simulink model "afe_dqctrl_inv_psm"  (R2026a)
settings: Solver=ode23t  StopTime=simlength  FixedStep=tc  MaxStep=glb_time.tc  RelTol=1e-4
values from neighbouring files (symbols this model uses):
  afe_ctrl = ctrl_afe_setup(glb_time.ts_afe, grid_emu.omega_grid_nom)    [init_model.m]
  afe_pwm_phase_shift_mod1 = 0    [init_model.m]
  CTRPIFF_CLIP_RELEASE = 0.001    [init_model.m]
  filters = setup_global_filters(glb_time.ts_afe, glb_time.ts_inv, glb_time.ts_dab, glb_time.tc)    [init_model.m]
  glb_time = timing_setup(fpwm_afe, trgo_afe, fpwm_inv, trgo_inv, fpwm_single_phase_inv, trgo_single_phase_inv, fpwm_dab, trgo_dab,      fpwm_psfbc, trgo_psfbc, fpwm_isop_rail, trgo_isop_rail, fpwm_cllc, trgo_cllc, t_measure, tc_factor, tc_decimation, delay_pwm, dead_time_afe,      dead_time_inv, dead_time_single_phase_inv, dead_time_dab, dead_time_psfbc, dead_time_isop_rail, dead_time_cllc)    [init_model.m]
  grid_emu = grid_three_phase_emulator('Dyn11', delta_star, grid_nominal_power, application_voltage, us1, us2, fgrid,                  eq_grid_inductance, eq_grid_resistance, eta, ucc, i1m, p_iron, n1, n2, core_area, core_length, mur,                  up_xi_pu_ref, up_eta_pu_ref, un_xi_pu_ref, un_eta_pu_ref)    [init_model.m]
  heatsink = liquid_cooled_plate_2kw_setup(weight, no_weight, cp_al, heat_capacity_hs, thermal_conductivity_al,      Rth_switch_HA, Rth_mosfet_HA, Rth_diode_HA, Tambient, DThs_init)    [init_model.m]
  inv_pwm_phase_shift_mod1 = 0    [init_model.m]
  ki_align = 18    [init_model.m]
  kp_align = 0.25    [init_model.m]
  lim_down_align = -0.05    [init_model.m]
  lim_up_align = 0.05    [init_model.m]
  omega_m_sim = psm.omega_m_bez    [init_model.m]
  psm = psm_calculus()    [init_model.m]
  psm_ctrl = ctrl_pmsm_setup(glb_time.ts_inv, psm.omega_bez, u_psm_scale, psm.Jm_norm)    [init_model.m]
  simlength = 1.75    [init_model.m]
  Tambient = 40    [init_model.m]
  time_gain_afe_module_1 = 1.0002    [init_model.m]
  time_gain_inv_module_2 = 1.001    [init_model.m]
  time_start_motor_control = 0.25    [init_model.m]
  torque_overload_factor = 1.15    [init_model.m]
  u_cm_comp_mod1 = 0    [init_model.m]
  u_psm_scale_ekf = sqrt(3)/2 * 2/3 * hwdata.inv.udc_nom/psm.ubez    [init_model.m]
undefined symbols (not defined in the file or in its folder): hwdata, igbt, magnitude, omega_m_bez, rpm_base, torque_base
libraries: fl_lib x99, nesl_utility x96, igbt_simple_lib x12, single_phase_transformer_lib x3, threephase_inductor_lib x2, dclink_for_two_levels x2, three_phase_pwm_modulator x2, cstblocks_lti x2, discrete_time_low_pass_filter x1, lithium_ion_battery x1, three_phase_voltage_with_frt_emulator x1, simple_flexible_shaft x1
(part 7 of 9)

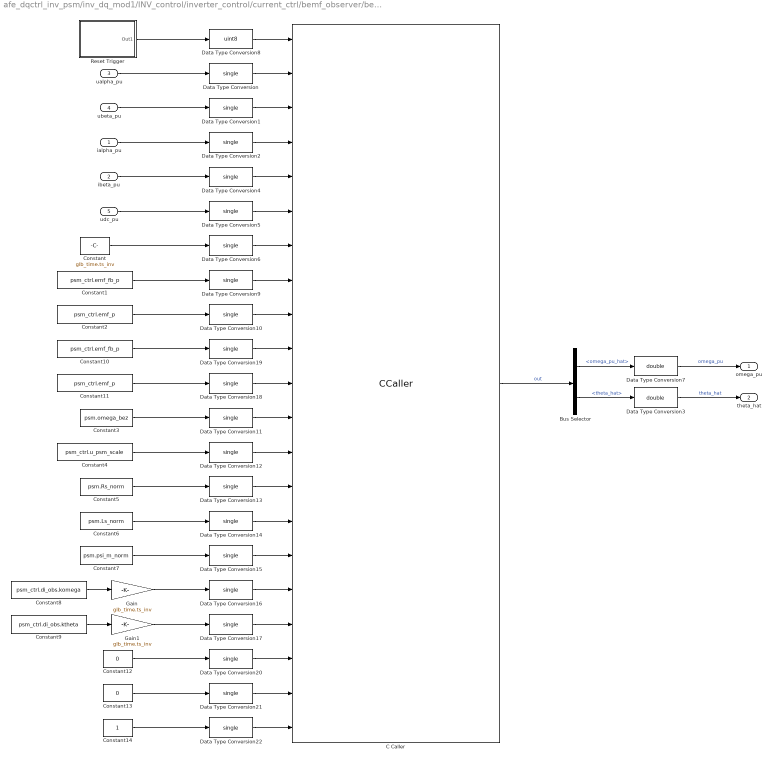
== system afe_dqctrl_inv_psm/inv_dq_mod1/INV_control/inverter_control/current_ctrl/bemf_observer/bemf_observer_ccaller ==
  ialpha_pu : Inport
  ibeta_pu : Inport  Port=2
  ualpha_pu : Inport  Port=3
  ubeta_pu : Inport  Port=4
  udc_pu : Inport  Port=5
  Bus Selector : BusSelector  OutputSignals=omega_pu_hat,theta_hat
  C Caller : CCaller  FunctionName=bemf_obsv_process_simulink  PortSpecificationStruct="%)30     .    N\"8   8    (     @         %    \"    !8    !     0         %  0 \"0    $    _    07)G3F%M90  4&]R=$YA;64 4V-O<&4     26YD97@     5'EP90      4VEZ90      27-';&]B86P   X    P    !@    @    $          4    (     0    ,    !         !   P!O=70 #@   #     &    \"     0         !0    @    !     P    $         $  # &]U=  .    .     8    (    !          %    \"     $    &     0         0  ...(+12985 chars)"
  Constant : Constant  Value=glb_time.ts_inv
  Constant1 : Constant  Value=psm_ctrl.emf_fb_p
  Constant10 : Constant  Value=psm_ctrl.emf_fb_p
  Constant11 : Constant  Value=psm_ctrl.emf_p
  Constant12 : Constant  Value=0
  Constant13 : Constant  Value=0
  Constant14 : Constant
  Constant2 : Constant  Value=psm_ctrl.emf_p
  Constant3 : Constant  Value=psm.omega_bez
  Constant4 : Constant  Value=psm_ctrl.u_psm_scale
  Constant5 : Constant  Value=psm.Rs_norm
  Constant6 : Constant  Value=psm.Ls_norm
  Constant7 : Constant  Value=psm.psi_m_norm
  Constant8 : Constant  Value=psm_ctrl.di_obs.komega
  Constant9 : Constant  Value=psm_ctrl.di_obs.ktheta
  Data Type Conversion{,1..2,4..6,9..22} (20 alike) : DataTypeConversion  OutDataTypeStr=single  SaturateOnIntegerOverflow=off  RndMeth=Floor
  Data Type Conversion3 : DataTypeConversion  OutDataTypeStr=double  SaturateOnIntegerOverflow=off  RndMeth=Floor
  Data Type Conversion7 : DataTypeConversion  OutDataTypeStr=double  SaturateOnIntegerOverflow=off  RndMeth=Floor
  Data Type Conversion8 : DataTypeConversion  OutDataTypeStr=uint8  SaturateOnIntegerOverflow=off  RndMeth=Floor
  Gain : Gain  Gain=glb_time.ts_inv
  Gain1 : Gain  Gain=glb_time.ts_inv
  Reset Trigger : Subsystem
  omega_pu : Outport
  theta_hat : Outport  Port=2
  wires:
  Data Type Conversion5/1 -> C Caller/6
  Data Type Conversion/1 -> C Caller/2
  C Caller/1 -> Bus Selector/1  "out"
  Data Type Conversion1/1 -> C Caller/3
  Data Type Conversion4/1 -> C Caller/5
  Data Type Conversion2/1 -> C Caller/4
  Data Type Conversion6/1 -> C Caller/7
  Bus Selector/2 -> Data Type Conversion3/1  "<theta_hat>"
  Bus Selector/1 -> Data Type Conversion7/1  "<omega_pu_hat>"
  Data Type Conversion7/1 -> omega_pu/1  "omega_pu"
  Data Type Conversion3/1 -> theta_hat/1  "theta_hat"
  Data Type Conversion8/1 -> C Caller/1
  Data Type Conversion9/1 -> C Caller/8
  Data Type Conversion10/1 -> C Caller/9
  Data Type Conversion19/1 -> C Caller/10
  Data Type Conversion18/1 -> C Caller/11
  Data Type Conversion11/1 -> C Caller/12
  Data Type Conversion12/1 -> C Caller/13
  Data Type Conversion13/1 -> C Caller/14
  Data Type Conversion14/1 -> C Caller/15
  Data Type Conversion15/1 -> C Caller/16
  Data Type Conversion16/1 -> C Caller/17
  Data Type Conversion17/1 -> C Caller/18
  Data Type Conversion20/1 -> C Caller/19
  Data Type Conversion21/1 -> C Caller/20
  Data Type Conversion22/1 -> C Caller/21
  Constant14/1 -> Data Type Conversion22/1
  Constant13/1 -> Data Type Conversion21/1
  Constant12/1 -> Data Type Conversion20/1
  Constant9/1 -> Gain1/1
  Constant8/1 -> Gain/1
  Constant7/1 -> Data Type Conversion15/1
  Constant6/1 -> Data Type Conversion14/1
  Constant5/1 -> Data Type Conversion13/1
  Constant4/1 -> Data Type Conversion12/1
  Constant3/1 -> Data Type Conversion11/1
  Constant11/1 -> Data Type Conversion18/1
  Constant10/1 -> Data Type Conversion19/1
  Constant2/1 -> Data Type Conversion10/1
  Constant1/1 -> Data Type Conversion9/1
  Constant/1 -> Data Type Conversion6/1
  ibeta_pu/1 -> Data Type Conversion4/1
  ialpha_pu/1 -> Data Type Conversion2/1
  ubeta_pu/1 -> Data Type Conversion1/1
  ualpha_pu/1 -> Data Type Conversion/1
  Reset Trigger/1(Out1) -> Data Type Conversion8/1
  udc_pu/1 -> Data Type Conversion5/1
  Gain/1 -> Data Type Conversion16/1
  Gain1/1 -> Data Type Conversion17/1

== system afe_dqctrl_inv_psm/inv_dq_mod1/INV_control/inverter_control/current_ctrl/current_ctrl/MTPA _mod1 ==
  iq_ref : Inport
  Gain1 : Gain  Gain=1/(psm.Ld_norm - psm.Lq_norm)/2
  Gain2 : Gain  Gain=1/(psm.Ld_norm - psm.Lq_norm)/2
  Gain3 : Gain  Gain=-1
  Math Function1 : Math  Operator=magnitude^2  SignedPower=on
  Math Function4 : Math  Operator=magnitude^2  SignedPower=on
  Sqrt : Sqrt
  Sum : Sum  Inputs=|++
  Sum1 : Sum  Inputs=|-+
  id_ref_pu < x < 0 : Saturate  UpperLimit=0  LowerLimit=-psm_ctrl.id_lim
  Id_ref_mtpa : Outport  VectorParamsAs1DForOutWhenUnconnected=off
  wires:
  Sum1/1 -> Gain3/1
  id_ref_pu < x < 0/1 -> Id_ref_mtpa/1
  Math Function4/1 -> Sum/1
  Math Function1/1 -> Sum/2
  Gain1/1 -> Math Function4/1
  Sum/1 -> Sqrt/1
  Sqrt/1 -> Sum1/2
  iq_ref/1 -> Math Function1/1
  Gain2/1 -> Sum1/1
  [motor_speed_pu_ctrl_mod1] -> Gain1/1, Gain2/1
  Gain3/1 -> id_ref_pu < x < 0/1

== system afe_dqctrl_inv_psm/inv_dq_mod1/INV_control/inverter_control/current_ctrl/current_ctrl/dq_pi_with_vector_antiwindup mod1 ==
  id_ref : Inport
  id : Inport  Port=2
  iq_ref : Inport  Port=3
  iq : Inport  Port=4
  udc_pu : Inport  Port=5
  Variant Source : VariantSource  VariantControls={use_current_controller_from_simulink_module_1 == 1, use_current_controller_from_ccaller_module_1 == 1}
  Variant Source1 : VariantSource  VariantControls={use_current_controller_from_simulink_module_1 == 1, use_current_controller_from_ccaller_module_1 == 1}
  dq_vector_pi : Subsystem
  dq_vector_pi_ccaller : Subsystem
  simulink/Ccaller VectorPI : Scope  NumInputPorts=2
      settings: ActiveDisplayYMinimum=-0.12579688616096973  ActiveDisplayYMaximum=0.43534495122730732
  ctrl_d_u : Outport
  ctrl_q_u : Outport  Port=2
  wires:
  id/1 -> dq_vector_pi_ccaller/1(id), dq_vector_pi/1(id)  "id"
  id_ref/1 -> dq_vector_pi_ccaller/2(id_ref), dq_vector_pi/2(id_ref)  "id_ref"
  iq/1 -> dq_vector_pi_ccaller/3(iq), dq_vector_pi/3(iq)  "iq"
  iq_ref/1 -> dq_vector_pi_ccaller/4(iq_ref), dq_vector_pi/4(iq_ref)  "iq_ref"
  dq_vector_pi/1(md_sat) -> Variant Source/1
  dq_vector_pi_ccaller/2(uq_ctrl_out) -> Variant Source1/2
  dq_vector_pi/2(mq_sat) -> Variant Source1/1
  dq_vector_pi_ccaller/1(ud_ctrl_out) -> Variant Source/2
  Variant Source/1 -> ctrl_d_u/1, simulink/Ccaller VectorPI/1  "ctrl_d_u"
  Variant Source1/1 -> simulink/Ccaller VectorPI/2, ctrl_q_u/1  "ctrl_q_u"
  udc_pu/1 -> dq_vector_pi_ccaller/5(udc_pu)

== system afe_dqctrl_inv_psm/inv_dq_mod1/INV_control/inverter_control/current_ctrl/current_ctrl/id_ref _mod1 ==
  id_mtpa : Inport
  Constant : Constant  Value=0
  Variant Source : VariantSource  VariantControls={use_mtpa == 1, use_mtpa == 0}
  id_ref : Outport
  wires:
  Variant Source/1 -> id_ref/1
  id_mtpa/1 -> Variant Source/1
  Constant/1 -> Variant Source/2

== system afe_dqctrl_inv_psm/inv_dq_mod1/INV_control/inverter_control/current_ctrl/current_ctrl/output voltage transformation ==
  Unit Delay2 : UnitDelay  SampleTime=-1
  Unit Delay3 : UnitDelay  SampleTime=-1
  dq2alphabeta : MATLAB Function  TreatAsAtomicUnit=on
  tag scope: ualpha_pu_mod1=scoped, ubeta_pu_mod1=scoped
  wires:
  [ud_pu_mod1] -> dq2alphabeta/1(d)
  [uq_pu_mod1] -> dq2alphabeta/2(q)
  Unit Delay2/1 -> [ualpha_pu_mod1]
  dq2alphabeta/2(beta) -> Unit Delay3/1
  Unit Delay3/1 -> [ubeta_pu_mod1]
  dq2alphabeta/1(alpha) -> Unit Delay2/1
  [motor_phase_ctrl_mod1] -> dq2alphabeta/3(gamma)

== system afe_dqctrl_inv_psm/inv_dq_mod1/INV_control/inverter_control/phase_compensation_1/alignment_ctrl/pi ==
  u_ref : Inport
  u : Inport  Port=2
  1/Ti : Gain  Gain=kp  SaturateOnIntegerOverflow=on  OutDataTypeStr=Inherit: Same as input  ParamDataTypeStr=Inherit: Same as input
  Saturation : Saturate  UpperLimit=lim_up  LowerLimit=lim_down
  Sum1 : Sum  Inputs=+++  SaturateOnIntegerOverflow=on
  Sum2 : Sum  Inputs=-+  SaturateOnIntegerOverflow=on
  Sum3 : Sum  Inputs=-+  SaturateOnIntegerOverflow=on
  Unit Delay4 : UnitDelay  SampleTime=-1
  kp : Gain  Gain=ki  SaturateOnIntegerOverflow=on  OutDataTypeStr=Inherit: Same as input  ParamDataTypeStr=Inherit: Same as input
  y : Outport
  wires:
  1/Ti/1 -> Sum1/1, Sum3/1
  kp/1 -> Sum1/2
  Sum3/1 -> Unit Delay4/1
  Unit Delay4/1 -> Sum1/3
  u_ref/1 -> Sum2/2
  u/1 -> Sum2/1
  Sum2/1 -> kp/1, 1/Ti/1
  Sum1/1 -> Saturation/1
  Saturation/1 -> Sum3/2, y/1

== system afe_dqctrl_inv_psm/inv_dq_mod1/inverter/inverter/three_phase_inverter_with_igbt_simple/three_phase_inverter_with_igbt_simple/igbt_simple_1 ==
  note: P_sw
  Capacitor : fl_lib/Electrical/Electrical Elements/Capacitor  c=Csnubber_m F  r=Rsnubber_m Ohm  g=0 1/Ohm  i_specify=off  i_priority=None  i=0 A  i_nominal_specify=off  i_nominal_value=1  i_nominal_unit=A  v_specify=off  v_priority=None  v=0 V  v_nominal_specify=off  v_nominal_value=1  v_nominal_unit=V  vc_specify=off  vc_priority=High  vc=0 V  vc_nominal_specify=off  vc_nominal_value=1  vc_nominal_unit=V
  IGBT_simple : Subsystem
      settings: PortSchema="{\"entries\":[{\"content\":{\"sides\":[{\"content\":{\"connectorIds\":[\"LConn1\"]},\"type\":\"ConnectorPlacement.EquallySpacedRectSide\",\"uuid\":\"c3d88d60-081d-4221-ab18-079856838dba\"},{\"content\":{\"side\":\"RIGHT\"},\"type\":\"ConnectorPlacement.EquallySpacedRectSide\",\"uuid\":\"76e7d76c-8b60-4107-8aac-a7654bd886e1\"},{\"content\":{\"connectorIds\":[\"LConn2\"],\"side\":\"TOP\"},\"type\":\"ConnectorPlacement.EquallySpacedRectSide\",\"uuid\":\"fbef57e1-7143-4076-ada8-0654b1d9ee0b\"},{\"content\":{\"connectorIds\":[\"RConn1\"],\"side\":\"BOTTOM\"},\"type\":\"ConnectorPlacement.EquallySpacedRectSide\",\"uuid\":\"f2fea5db-9515-452a-a480-7d54bae36c49\"}]},\"type\":\"ConnectorPlacement.EquallySpacedConnector\",\"uuid\":\"cddff0b8-236e-4840-ad87-03abcdd65fe7\"}],\"packageUris\":[\"http://schema.mathworks.com/mf0/Connector/R2020b\"],\"version\":\"1.0\"}"
  Voltage Sensor : fl_lib/Electrical/Electrical Sensors/Voltage Sensor
  uph : nesl_utility/PS-Simulink Converter  PhysicalDomain=network_engine_domain  SubClassName=ps_output  LeftPortType=input  RightPortType=output  PseudoPeriodic=off  Frequencies=[]  VectorFormat=1-D array  Unit=V  AffineConversion=off
  G : PMIOPort  Side=Left
  C : PMIOPort  Port=2  Side=Left
  E : PMIOPort  Port=3  Side=Right
  tag scope: igbt_voltage_Q1=scoped
  wires:
  uph/1 -> [igbt_voltage_Q1]  "uph"
  connections:
  G/RConn1 -- IGBT_simple/LConn1
  Voltage Sensor/RConn1 -- uph/LConn1
  Capacitor/LConn1 -- Voltage Sensor/LConn1 -- C/RConn1 -- IGBT_simple/LConn2
  Capacitor/RConn1 -- Voltage Sensor/RConn2 -- E/RConn1 -- IGBT_simple/RConn1

== system afe_dqctrl_inv_psm/inv_dq_mod1/inverter/inverter/three_phase_inverter_with_igbt_simple/three_phase_inverter_with_igbt_simple/igbt_simple_2 ==
  Capacitor : fl_lib/Electrical/Electrical Elements/Capacitor  c=Csnubber_m F  r=Rsnubber_m Ohm  g=0 1/Ohm  i_specify=off  i_priority=None  i=0 A  i_nominal_specify=off  i_nominal_value=1  i_nominal_unit=A  v_specify=off  v_priority=None  v=0 V  v_nominal_specify=off  v_nominal_value=1  v_nominal_unit=V  vc_specify=off  vc_priority=High  vc=0 V  vc_nominal_specify=off  vc_nominal_value=1  vc_nominal_unit=V
  IGBT_simple : Subsystem
      settings: PortSchema="{\"entries\":[{\"content\":{\"sides\":[{\"content\":{\"connectorIds\":[\"LConn1\"]},\"type\":\"ConnectorPlacement.EquallySpacedRectSide\",\"uuid\":\"c3d88d60-081d-4221-ab18-079856838dba\"},{\"content\":{\"side\":\"RIGHT\"},\"type\":\"ConnectorPlacement.EquallySpacedRectSide\",\"uuid\":\"76e7d76c-8b60-4107-8aac-a7654bd886e1\"},{\"content\":{\"connectorIds\":[\"LConn2\"],\"side\":\"TOP\"},\"type\":\"ConnectorPlacement.EquallySpacedRectSide\",\"uuid\":\"fbef57e1-7143-4076-ada8-0654b1d9ee0b\"},{\"content\":{\"connectorIds\":[\"RConn1\"],\"side\":\"BOTTOM\"},\"type\":\"ConnectorPlacement.EquallySpacedRectSide\",\"uuid\":\"f2fea5db-9515-452a-a480-7d54bae36c49\"}]},\"type\":\"ConnectorPlacement.EquallySpacedConnector\",\"uuid\":\"cddff0b8-236e-4840-ad87-03abcdd65fe7\"}],\"packageUris\":[\"http://schema.mathworks.com/mf0/Connector/R2020b\"],\"version\":\"1.0\"}"
  Voltage Sensor : fl_lib/Electrical/Electrical Sensors/Voltage Sensor
  uph : nesl_utility/PS-Simulink Converter  PhysicalDomain=network_engine_domain  SubClassName=ps_output  LeftPortType=input  RightPortType=output  PseudoPeriodic=off  Frequencies=[]  VectorFormat=1-D array  Unit=V  AffineConversion=off
  G : PMIOPort  Side=Left
  C : PMIOPort  Port=2  Side=Left
  E : PMIOPort  Port=3  Side=Right
  tag scope: igbt_voltage_Q2=scoped
  wires:
  uph/1 -> [igbt_voltage_Q2]  "uph"
  connections:
  Capacitor/RConn1 -- Voltage Sensor/RConn2 -- E/RConn1 -- IGBT_simple/RConn1
  Capacitor/LConn1 -- Voltage Sensor/LConn1 -- C/RConn1 -- IGBT_simple/LConn2
  Voltage Sensor/RConn1 -- uph/LConn1
  IGBT_simple/LConn1 -- G/RConn1

== system afe_dqctrl_inv_psm/inv_dq_mod1/inverter/inverter/three_phase_inverter_with_igbt_simple/three_phase_inverter_with_igbt_simple/igbt_simple_3 ==
  Capacitor : fl_lib/Electrical/Electrical Elements/Capacitor  c=Csnubber_m F  r=Rsnubber_m Ohm  g=0 1/Ohm  i_specify=off  i_priority=None  i=0 A  i_nominal_specify=off  i_nominal_value=1  i_nominal_unit=A  v_specify=off  v_priority=None  v=0 V  v_nominal_specify=off  v_nominal_value=1  v_nominal_unit=V  vc_specify=off  vc_priority=High  vc=0 V  vc_nominal_specify=off  vc_nominal_value=1  vc_nominal_unit=V
  IGBT_simple : Subsystem
      settings: PortSchema="{\"entries\":[{\"content\":{\"sides\":[{\"content\":{\"connectorIds\":[\"LConn1\"]},\"type\":\"ConnectorPlacement.EquallySpacedRectSide\",\"uuid\":\"c3d88d60-081d-4221-ab18-079856838dba\"},{\"content\":{\"side\":\"RIGHT\"},\"type\":\"ConnectorPlacement.EquallySpacedRectSide\",\"uuid\":\"76e7d76c-8b60-4107-8aac-a7654bd886e1\"},{\"content\":{\"connectorIds\":[\"LConn2\"],\"side\":\"TOP\"},\"type\":\"ConnectorPlacement.EquallySpacedRectSide\",\"uuid\":\"fbef57e1-7143-4076-ada8-0654b1d9ee0b\"},{\"content\":{\"connectorIds\":[\"RConn1\"],\"side\":\"BOTTOM\"},\"type\":\"ConnectorPlacement.EquallySpacedRectSide\",\"uuid\":\"f2fea5db-9515-452a-a480-7d54bae36c49\"}]},\"type\":\"ConnectorPlacement.EquallySpacedConnector\",\"uuid\":\"cddff0b8-236e-4840-ad87-03abcdd65fe7\"}],\"packageUris\":[\"http://schema.mathworks.com/mf0/Connector/R2020b\"],\"version\":\"1.0\"}"
  Voltage Sensor : fl_lib/Electrical/Electrical Sensors/Voltage Sensor
  uph : nesl_utility/PS-Simulink Converter  PhysicalDomain=network_engine_domain  SubClassName=ps_output  LeftPortType=input  RightPortType=output  PseudoPeriodic=off  Frequencies=[]  VectorFormat=1-D array  Unit=V  AffineConversion=off
  G : PMIOPort  Side=Left
  C : PMIOPort  Port=2  Side=Left
  E : PMIOPort  Port=3  Side=Right
  tag scope: igbt_voltage_Q3=scoped
  wires:
  uph/1 -> [igbt_voltage_Q3]  "uph"
  connections:
  IGBT_simple/LConn1 -- G/RConn1
  Voltage Sensor/RConn1 -- uph/LConn1
  Voltage Sensor/LConn1 -- Capacitor/LConn1 -- C/RConn1 -- IGBT_simple/LConn2
  Voltage Sensor/RConn2 -- Capacitor/RConn1 -- E/RConn1 -- IGBT_simple/RConn1

== system afe_dqctrl_inv_psm/inv_dq_mod1/inverter/inverter/three_phase_inverter_with_igbt_simple/three_phase_inverter_with_igbt_simple/igbt_simple_4 ==
  Capacitor : fl_lib/Electrical/Electrical Elements/Capacitor  c=Csnubber_m F  r=Rsnubber_m Ohm  g=0 1/Ohm  i_specify=off  i_priority=None  i=0 A  i_nominal_specify=off  i_nominal_value=1  i_nominal_unit=A  v_specify=off  v_priority=None  v=0 V  v_nominal_specify=off  v_nominal_value=1  v_nominal_unit=V  vc_specify=off  vc_priority=High  vc=0 V  vc_nominal_specify=off  vc_nominal_value=1  vc_nominal_unit=V
  IGBT_simple : Subsystem
      settings: PortSchema="{\"entries\":[{\"content\":{\"sides\":[{\"content\":{\"connectorIds\":[\"LConn1\"]},\"type\":\"ConnectorPlacement.EquallySpacedRectSide\",\"uuid\":\"c3d88d60-081d-4221-ab18-079856838dba\"},{\"content\":{\"side\":\"RIGHT\"},\"type\":\"ConnectorPlacement.EquallySpacedRectSide\",\"uuid\":\"76e7d76c-8b60-4107-8aac-a7654bd886e1\"},{\"content\":{\"connectorIds\":[\"LConn2\"],\"side\":\"TOP\"},\"type\":\"ConnectorPlacement.EquallySpacedRectSide\",\"uuid\":\"fbef57e1-7143-4076-ada8-0654b1d9ee0b\"},{\"content\":{\"connectorIds\":[\"RConn1\"],\"side\":\"BOTTOM\"},\"type\":\"ConnectorPlacement.EquallySpacedRectSide\",\"uuid\":\"f2fea5db-9515-452a-a480-7d54bae36c49\"}]},\"type\":\"ConnectorPlacement.EquallySpacedConnector\",\"uuid\":\"cddff0b8-236e-4840-ad87-03abcdd65fe7\"}],\"packageUris\":[\"http://schema.mathworks.com/mf0/Connector/R2020b\"],\"version\":\"1.0\"}"
  Voltage Sensor : fl_lib/Electrical/Electrical Sensors/Voltage Sensor
  uph : nesl_utility/PS-Simulink Converter  PhysicalDomain=network_engine_domain  SubClassName=ps_output  LeftPortType=input  RightPortType=output  PseudoPeriodic=off  Frequencies=[]  VectorFormat=1-D array  Unit=V  AffineConversion=off
  G : PMIOPort  Side=Left
  C : PMIOPort  Port=2  Side=Left
  E : PMIOPort  Port=3  Side=Right
  tag scope: igbt_voltage_Q4=scoped
  wires:
  uph/1 -> [igbt_voltage_Q4]  "uph"
  connections:
  Capacitor/RConn1 -- Voltage Sensor/RConn2 -- E/RConn1 -- IGBT_simple/RConn1
  Capacitor/LConn1 -- Voltage Sensor/LConn1 -- C/RConn1 -- IGBT_simple/LConn2
  Voltage Sensor/RConn1 -- uph/LConn1
  IGBT_simple/LConn1 -- G/RConn1

== system afe_dqctrl_inv_psm/inv_dq_mod1/inverter/inverter/three_phase_inverter_with_igbt_simple/three_phase_inverter_with_igbt_simple/igbt_simple_5 ==
  Capacitor : fl_lib/Electrical/Electrical Elements/Capacitor  c=Csnubber_m F  r=Rsnubber_m Ohm  g=0 1/Ohm  i_specify=off  i_priority=None  i=0 A  i_nominal_specify=off  i_nominal_value=1  i_nominal_unit=A  v_specify=off  v_priority=None  v=0 V  v_nominal_specify=off  v_nominal_value=1  v_nominal_unit=V  vc_specify=off  vc_priority=High  vc=0 V  vc_nominal_specify=off  vc_nominal_value=1  vc_nominal_unit=V
  IGBT_simple : Subsystem
      settings: PortSchema="{\"entries\":[{\"content\":{\"sides\":[{\"content\":{\"connectorIds\":[\"LConn1\"]},\"type\":\"ConnectorPlacement.EquallySpacedRectSide\",\"uuid\":\"c3d88d60-081d-4221-ab18-079856838dba\"},{\"content\":{\"side\":\"RIGHT\"},\"type\":\"ConnectorPlacement.EquallySpacedRectSide\",\"uuid\":\"76e7d76c-8b60-4107-8aac-a7654bd886e1\"},{\"content\":{\"connectorIds\":[\"LConn2\"],\"side\":\"TOP\"},\"type\":\"ConnectorPlacement.EquallySpacedRectSide\",\"uuid\":\"fbef57e1-7143-4076-ada8-0654b1d9ee0b\"},{\"content\":{\"connectorIds\":[\"RConn1\"],\"side\":\"BOTTOM\"},\"type\":\"ConnectorPlacement.EquallySpacedRectSide\",\"uuid\":\"f2fea5db-9515-452a-a480-7d54bae36c49\"}]},\"type\":\"ConnectorPlacement.EquallySpacedConnector\",\"uuid\":\"cddff0b8-236e-4840-ad87-03abcdd65fe7\"}],\"packageUris\":[\"http://schema.mathworks.com/mf0/Connector/R2020b\"],\"version\":\"1.0\"}"
  Voltage Sensor : fl_lib/Electrical/Electrical Sensors/Voltage Sensor
  uph : nesl_utility/PS-Simulink Converter  PhysicalDomain=network_engine_domain  SubClassName=ps_output  LeftPortType=input  RightPortType=output  PseudoPeriodic=off  Frequencies=[]  VectorFormat=1-D array  Unit=V  AffineConversion=off
  G : PMIOPort  Side=Left
  C : PMIOPort  Port=2  Side=Left
  E : PMIOPort  Port=3  Side=Right
  tag scope: igbt_voltage_Q5=scoped
  wires:
  uph/1 -> [igbt_voltage_Q5]  "uph"
  connections:
  IGBT_simple/LConn1 -- G/RConn1
  Voltage Sensor/RConn1 -- uph/LConn1
  Voltage Sensor/LConn1 -- Capacitor/LConn1 -- C/RConn1 -- IGBT_simple/LConn2
  Voltage Sensor/RConn2 -- Capacitor/RConn1 -- E/RConn1 -- IGBT_simple/RConn1

== system afe_dqctrl_inv_psm/inv_dq_mod1/inverter/inverter/three_phase_inverter_with_igbt_simple/three_phase_inverter_with_igbt_simple/igbt_simple_6 ==
  Capacitor : fl_lib/Electrical/Electrical Elements/Capacitor  c=Csnubber_m F  r=Rsnubber_m Ohm  g=0 1/Ohm  i_specify=off  i_priority=None  i=0 A  i_nominal_specify=off  i_nominal_value=1  i_nominal_unit=A  v_specify=off  v_priority=None  v=0 V  v_nominal_specify=off  v_nominal_value=1  v_nominal_unit=V  vc_specify=off  vc_priority=High  vc=0 V  vc_nominal_specify=off  vc_nominal_value=1  vc_nominal_unit=V
  IGBT_simple : Subsystem
      settings: PortSchema="{\"entries\":[{\"content\":{\"sides\":[{\"content\":{\"connectorIds\":[\"LConn1\"]},\"type\":\"ConnectorPlacement.EquallySpacedRectSide\",\"uuid\":\"c3d88d60-081d-4221-ab18-079856838dba\"},{\"content\":{\"side\":\"RIGHT\"},\"type\":\"ConnectorPlacement.EquallySpacedRectSide\",\"uuid\":\"76e7d76c-8b60-4107-8aac-a7654bd886e1\"},{\"content\":{\"connectorIds\":[\"LConn2\"],\"side\":\"TOP\"},\"type\":\"ConnectorPlacement.EquallySpacedRectSide\",\"uuid\":\"fbef57e1-7143-4076-ada8-0654b1d9ee0b\"},{\"content\":{\"connectorIds\":[\"RConn1\"],\"side\":\"BOTTOM\"},\"type\":\"ConnectorPlacement.EquallySpacedRectSide\",\"uuid\":\"f2fea5db-9515-452a-a480-7d54bae36c49\"}]},\"type\":\"ConnectorPlacement.EquallySpacedConnector\",\"uuid\":\"cddff0b8-236e-4840-ad87-03abcdd65fe7\"}],\"packageUris\":[\"http://schema.mathworks.com/mf0/Connector/R2020b\"],\"version\":\"1.0\"}"
  Voltage Sensor : fl_lib/Electrical/Electrical Sensors/Voltage Sensor
  uph : nesl_utility/PS-Simulink Converter  PhysicalDomain=network_engine_domain  SubClassName=ps_output  LeftPortType=input  RightPortType=output  PseudoPeriodic=off  Frequencies=[]  VectorFormat=1-D array  Unit=V  AffineConversion=off
  G : PMIOPort  Side=Left
  C : PMIOPort  Port=2  Side=Left
  E : PMIOPort  Port=3  Side=Right
  tag scope: igbt_voltage_Q6=scoped
  wires:
  uph/1 -> [igbt_voltage_Q6]  "uph"
  connections:
  Capacitor/RConn1 -- Voltage Sensor/RConn2 -- E/RConn1 -- IGBT_simple/RConn1
  Capacitor/LConn1 -- Voltage Sensor/LConn1 -- C/RConn1 -- IGBT_simple/LConn2
  Voltage Sensor/RConn1 -- uph/LConn1
  IGBT_simple/LConn1 -- G/RConn1

== system afe_dqctrl_inv_psm/inv_dq_mod1/inverter/inverter/three_phase_inverter_with_igbt_simple/three_phase_inverter_with_igbt_simple/module_1 ==
  Bus Creator : BusCreator  Inputs=18
  m : Outport
  wires:
  [diode_HA_temp_Q1] -> Bus Creator/8  "diode_HA_temp_Q1"
  [igbt_voltage_Q2] -> Bus Creator/10  "igbt_voltage_Q2"
  [igbt_voltage_Q1] -> Bus Creator/2  "igbt_voltage_Q1"
  [igbt_ploss_Q2] -> Bus Creator/9  "igbt_ploss_Q2"
  [igbt_current_Q2] -> Bus Creator/11  "igbt_current_Q2"
  [diode_ploss_Q1] -> Bus Creator/6  "diode_ploss_Q1"
  [diode_JH_temp_Q1] -> Bus Creator/7  "diode_JH_temp_Q1"
  [igbt_HA_temp_Q1] -> Bus Creator/5  "igbt_HA_temp_Q1"
  [igbt_ploss_Q1] -> Bus Creator/1  "igbt_ploss_Q1"
  [diode_JH_temp_Q2] -> Bus Creator/15  "diode_JH_temp_Q2"
  [diode_HA_temp_Q2] -> Bus Creator/16  "diode_HA_temp_Q2"
  [diode_ploss_Q2] -> Bus Creator/14  "diode_ploss_Q2"
  [igbt_HA_temp_Q2] -> Bus Creator/13  "igbt_HA_temp_Q2"
  [igbt_JH_temp_Q2] -> Bus Creator/12  "igbt_JH_temp_Q2"
  [igbt_JH_temp_Q1] -> Bus Creator/4  "igbt_JH_temp_Q1"
  [igbt_current_Q1] -> Bus Creator/3  "igbt_current_Q1"
  Bus Creator/1 -> m/1  "module_1"
  [diode_current_Q1] -> Bus Creator/17  "diode_current_Q1"
  [diode_current_Q2] -> Bus Creator/18  "diode_current_Q2"

== system afe_dqctrl_inv_psm/inv_dq_mod1/inverter/inverter/three_phase_inverter_with_igbt_simple/three_phase_inverter_with_igbt_simple/module_2 ==
  Bus Creator1 : BusCreator  Inputs=18
  m : Outport
  wires:
  [diode_HA_temp_Q4] -> Bus Creator1/16  "diode_HA_temp_Q4"
  [igbt_HA_temp_Q3] -> Bus Creator1/5  "igbt_HA_temp_Q3"
  [igbt_JH_temp_Q3] -> Bus Creator1/4  "igbt_JH_temp_Q3"
  [diode_ploss_Q3] -> Bus Creator1/6  "diode_ploss_Q3"
  [diode_JH_temp_Q4] -> Bus Creator1/15  "diode_JH_temp_Q4"
  [igbt_ploss_Q3] -> Bus Creator1/1  "igbt_ploss_Q3"
  [igbt_JH_temp_Q4] -> Bus Creator1/12  "igbt_JH_temp_Q4"
  [igbt_voltage_Q3] -> Bus Creator1/2  "igbt_voltage_Q3"
  [igbt_current_Q4] -> Bus Creator1/11  "igbt_current_Q4"
  [diode_HA_temp_Q3] -> Bus Creator1/8  "diode_HA_temp_Q3"
  [igbt_voltage_Q4] -> Bus Creator1/10  "igbt_voltage_Q4"
  [igbt_ploss_Q4] -> Bus Creator1/9  "igbt_ploss_Q4"
  [igbt_HA_temp_Q4] -> Bus Creator1/13  "igbt_HA_temp_Q4"
  [diode_JH_temp_Q3] -> Bus Creator1/7  "diode_JH_temp_Q3"
  [diode_ploss_Q4] -> Bus Creator1/14  "diode_ploss_Q4"
  [igbt_current_Q3] -> Bus Creator1/3  "igbt_current_Q3"
  Bus Creator1/1 -> m/1  "module_2"
  [diode_current_Q4] -> Bus Creator1/18  "diode_current_Q4"
  [diode_current_Q3] -> Bus Creator1/17  "diode_current_Q3"

== system afe_dqctrl_inv_psm/inv_dq_mod1/inverter/inverter/three_phase_inverter_with_igbt_simple/three_phase_inverter_with_igbt_simple/module_3 ==
  Bus Creator1 : BusCreator  Inputs=18
  m : Outport
  wires:
  [diode_ploss_Q6] -> Bus Creator1/14  "diode_ploss_Q6"
  [igbt_HA_temp_Q5] -> Bus Creator1/5  "igbt_HA_temp_Q5"
  [igbt_voltage_Q6] -> Bus Creator1/10  "igbt_voltage_Q6"
  [igbt_voltage_Q5] -> Bus Creator1/2  "igbt_voltage_Q5"
  [igbt_JH_temp_Q6] -> Bus Creator1/12  "igbt_JH_temp_Q6"
  [igbt_current_Q6] -> Bus Creator1/11  "igbt_current_Q6"
  [diode_JH_temp_Q6] -> Bus Creator1/15  "diode_JH_temp_Q6"
  [diode_HA_temp_Q5] -> Bus Creator1/8  "diode_HA_temp_Q5"
  [igbt_ploss_Q5] -> Bus Creator1/1  "igbt_ploss_Q5"
  [igbt_ploss_Q6] -> Bus Creator1/9  "igbt_ploss_Q6"
  [igbt_current_Q5] -> Bus Creator1/3  "igbt_current_Q5"
  [diode_JH_temp_Q5] -> Bus Creator1/7  "diode_JH_temp_Q5"
  [igbt_JH_temp_Q5] -> Bus Creator1/4  "igbt_JH_temp_Q5"
  [diode_HA_temp_Q6] -> Bus Creator1/16  "diode_HA_temp_Q6"
  [igbt_HA_temp_Q6] -> Bus Creator1/13  "igbt_HA_temp_Q6"
  [diode_ploss_Q5] -> Bus Creator1/6  "diode_ploss_Q5"
  Bus Creator1/1 -> m/1  "module_3"
  [diode_current_Q6] -> Bus Creator1/18  "diode_current_Q6"
  [diode_current_Q5] -> Bus Creator1/17  "diode_current_Q5"

== system afe_dqctrl_inv_psm/afe_dq_mod1/AFE_control/afe_control/acquisitions/phase_compensation_1/alignment_eval_afe1/pi ==
  u_ref : Inport
  u : Inport  Port=2
  1/Ti : Gain  Gain=kp  SaturateOnIntegerOverflow=on  OutDataTypeStr=Inherit: Same as input  ParamDataTypeStr=Inherit: Same as input
  Saturation : Saturate  UpperLimit=lim_up  LowerLimit=lim_down
  Sum1 : Sum  Inputs=+++  SaturateOnIntegerOverflow=on
  Sum2 : Sum  Inputs=-+  SaturateOnIntegerOverflow=on
  Sum3 : Sum  Inputs=-+  SaturateOnIntegerOverflow=on
  Unit Delay4 : UnitDelay  SampleTime=-1
  kp : Gain  Gain=ki  SaturateOnIntegerOverflow=on  OutDataTypeStr=Inherit: Same as input  ParamDataTypeStr=Inherit: Same as input
  y : Outport
  wires:
  1/Ti/1 -> Sum1/1, Sum3/1
  kp/1 -> Sum1/2
  Sum3/1 -> Unit Delay4/1
  Unit Delay4/1 -> Sum1/3
  u_ref/1 -> Sum2/2
  u/1 -> Sum2/1
  Sum2/1 -> kp/1, 1/Ti/1
  Sum1/1 -> Saturation/1
  Saturation/1 -> Sum3/2, y/1

== system afe_dqctrl_inv_psm/afe_dq_mod1/AFE_control/afe_control/grid_voltage_phase_lock_loops/FHT-PLL/pll_stageA/filter_and_transformation ==
  ug_a : Inport
  ug_b : Inport  Port=2
  ug_c : Inport  Port=3
  Bus Creator : BusCreator  Inputs=2
  Bus Creator1 : BusCreator  Inputs=3
  Bus Creator2 : BusCreator  Inputs=2
  Bus Creator3 : BusCreator  Inputs=3
  Bus Creator4 : BusCreator  Inputs=3
  FHTalpha : Subsystem
  FHTbeta : Subsystem
  FHTdqPLL : Scope  NumInputPorts=2
      settings: ActiveDisplayYMinimum=-1.5258214459194912  ActiveDisplayYMaximum=1.5258228058860459  DataLoggingVariableName=ScopeData12
  Gain : Gain  Gain=-1/2
  Gain1 : Gain  Gain=-1/2
  Sum : Sum  Inputs=|++
  Sum1 : Sum  Inputs=-+|
  To Workspace1 : ToWorkspace  VariableName=ugd_alpha_sim  SampleTime=-1
      settings: MaxDataPoints=glb_time.Ns_afe
  To Workspace2 : ToWorkspace  VariableName=ugd_beta_sim  SampleTime=-1
      settings: MaxDataPoints=glb_time.Ns_afe
  To Workspace3 : ToWorkspace  VariableName=u_fht_alpha_sim  SampleTime=-1
      settings: MaxDataPoints=glb_time.Ns_afe
  To Workspace4 : ToWorkspace  VariableName=v_fht_alpha_sim  SampleTime=-1
      settings: MaxDataPoints=glb_time.Ns_afe
  To Workspace5 : ToWorkspace  VariableName=u_fhtsr_alpha_sim  SampleTime=-1
      settings: MaxDataPoints=glb_time.Ns_afe
  To Workspace6 : ToWorkspace  VariableName=u_fhtsr_beta_sim  SampleTime=-1
      settings: MaxDataPoints=glb_time.Ns_afe
  To Workspace7 : ToWorkspace  VariableName=u_fht_beta_sim  SampleTime=-1
      settings: MaxDataPoints=glb_time.Ns_afe
  To Workspace8 : ToWorkspace  VariableName=v_fht_beta_sim  SampleTime=-1
      settings: MaxDataPoints=glb_time.Ns_afe
  To Workspace9 : ToWorkspace  VariableName=ugd_abc_grid_sim  SampleTime=-1
      settings: MaxDataPoints=glb_time.Ns_afe
  abc2alphabeta : MATLAB Function  TreatAsAtomicUnit=on
  grid_voltages : Scope  NumInputPorts=3
      settings: ActiveDisplayYMinimum=-1.3618303835391998  ActiveDisplayYMaximum=1.3331545889377594  DataLoggingVariableName=ScopeData13
  ug_alpha : Outport  VectorParamsAs1DForOutWhenUnconnected=off
  ug_beta : Outport  Port=2  VectorParamsAs1DForOutWhenUnconnected=off
  wires:
  ug_b/1 -> Bus Creator3/2, grid_voltages/2, abc2alphabeta/2(b)  "ugd_b"
  ug_c/1 -> Bus Creator3/3, grid_voltages/3, abc2alphabeta/3(c)  "ugd_c"
  ug_a/1 -> Bus Creator3/1, grid_voltages/1, abc2alphabeta/1(a)  "ugd_a"
  abc2alphabeta/1(alpha) -> To Workspace1/1, FHTalpha/1(u), Bus Creator4/1  "u_grid_alpha"
  abc2alphabeta/2(beta) -> FHTbeta/1(u), To Workspace2/1, Bus Creator1/1  "u_grid_beta"
  FHTalpha/1(ud_hat) -> To Workspace3/1, Bus Creator/1, Sum/1  "u_fht_alpha"
  Sum/1 -> Gain/1
  FHTbeta/1(ud_hat) -> Sum1/2, To Workspace7/1, Bus Creator2/1  "u_fht_beta"
  Sum1/1 -> Gain1/1
  Gain1/1 -> Bus Creator1/3, To Workspace6/1, ug_beta/1  "u_fhtsr_beta"
  Gain/1 -> Bus Creator4/3, To Workspace5/1, ug_alpha/1  "u_fhtsr_alpha"
  FHTbeta/2(uq_hat) -> Sum/2, To Workspace8/1, Bus Creator2/2  "v_fht_beta"
  FHTalpha/2(uq_hat) -> Sum1/1, To Workspace4/1, Bus Creator/2  "v_fht_alpha"
  Bus Creator1/1 -> FHTdqPLL/2
  Bus Creator4/1 -> FHTdqPLL/1
  Bus Creator/1 -> Bus Creator4/2  "FHTalpha"
  Bus Creator2/1 -> Bus Creator1/2  "FHTbeta"
  Bus Creator3/1 -> To Workspace9/1

== system afe_dqctrl_inv_psm/afe_dq_mod1/AFE_control/afe_control/grid_voltage_phase_lock_loops/FHT-PLL/pll_stageA/sequences ==
  u_grid_alpha : Inport
  u_grid_beta : Inport  Port=2
  phase_angle : Inport  Port=3
  alphabeta2xieta : MATLAB Function  TreatAsAtomicUnit=on
  u_grid_xi : Outport
  u_grid_eta : Outport  Port=2
  wires:
  alphabeta2xieta/1(xi) -> u_grid_xi/1  "u_grid_xi"
  alphabeta2xieta/2(eta) -> u_grid_eta/1  "u_grid_eta"
  u_grid_alpha/1 -> alphabeta2xieta/1(alpha)  "u_grid_alpha"
  u_grid_beta/1 -> alphabeta2xieta/2(beta)  "u_grid_beta"
  phase_angle/1 -> alphabeta2xieta/3(gamma)  "phase_angle"

== system afe_dqctrl_inv_psm/afe_dq_mod1/AFE_control/afe_control/grid_voltage_phase_lock_loops/FHT-PLL/pll_stageB/double_integrator_observer ==
  theta : Inport
  Gain : Gain  Gain=afe_ctrl.di_obs.Ldso  Multiplication=Matrix(K*u)
  Gain1 : Gain  Gain=afe_ctrl.di_obs.Adso  Multiplication=Matrix(K*u)
  Gain2 : Gain  Gain=afe_ctrl.di_obs.Cso  Multiplication=Matrix(K*u)
  Selector : Selector  InputPortWidth=2  IndexOptions=Index vector (dialog)  Indices=2  OutputSizes=1
  Sum : Sum  Inputs=-+|
  Sum1 : Sum  Inputs=|++
  Unit Delay : UnitDelay  SampleTime=-1
  bounder1 : MATLAB Function  TreatAsAtomicUnit=on
  bounder2 : MATLAB Function  TreatAsAtomicUnit=on
  omega_hat : Outport
  wires:
  Gain/1 -> Sum1/1
  Selector/1 -> omega_hat/1
  Gain2/1 -> bounder2/1(u)  "theta_hat"
  Gain1/1 -> Sum1/2
  Sum1/1 -> Unit Delay/1
  Sum/1 -> bounder1/1(u)  "e"
  Unit Delay/1 -> Gain1/1, Selector/1, Gain2/1
  theta/1 -> Sum/2  "theta"
  bounder1/1(y) -> Gain/1
  bounder2/1(y) -> Sum/1  "theta_hat_bounded"

== system afe_dqctrl_inv_psm/afe_dq_mod1/AFE_control/afe_control/grid_voltage_phase_lock_loops/FHT-PLL_simulink/pll_stageA/filter_and_transformation ==
  ug_a : Inport
  ug_b : Inport  Port=2
  ug_c : Inport  Port=3
  Bus Creator : BusCreator  Inputs=2
  Bus Creator1 : BusCreator  Inputs=3
  Bus Creator2 : BusCreator  Inputs=2
  Bus Creator4 : BusCreator  Inputs=3
  FHTalpha : Subsystem
  FHTbeta : Subsystem
  FHTdqPLL : Scope  NumInputPorts=2
      settings: ActiveDisplayYMinimum=-1.5258214459194912  ActiveDisplayYMaximum=1.5258228058860459  DataLoggingVariableName=ScopeData12
  Gain : Gain  Gain=-1/2
  Gain1 : Gain  Gain=-1/2
  Sum : Sum  Inputs=|++
  Sum1 : Sum  Inputs=-+|
  abc2alphabeta : MATLAB Function  TreatAsAtomicUnit=on
  grid_voltages : Scope  NumInputPorts=3
      settings: ActiveDisplayYMinimum=-1.3618303835391998  ActiveDisplayYMaximum=1.3331545889377594  DataLoggingVariableName=ScopeData13
  ug_alpha : Outport  VectorParamsAs1DForOutWhenUnconnected=off
  ug_beta : Outport  Port=2  VectorParamsAs1DForOutWhenUnconnected=off
  wires:
  Bus Creator2/1 -> Bus Creator1/2  "FHTbeta"
  Bus Creator/1 -> Bus Creator4/2  "FHTalpha"
  Bus Creator4/1 -> FHTdqPLL/1
  Bus Creator1/1 -> FHTdqPLL/2
  FHTalpha/2(ubeta) -> Bus Creator/2, Sum1/1  "v_fht_alpha"
  FHTbeta/2(ubeta) -> Bus Creator2/2, Sum/2  "v_fht_beta"
  Gain/1 -> ug_alpha/1, Bus Creator4/3  "u_fhtsr_alpha"
  Gain1/1 -> ug_beta/1, Bus Creator1/3  "u_fhtsr_beta"
  Sum1/1 -> Gain1/1
  FHTbeta/1(ualpha) -> Bus Creator2/1, Sum1/2  "u_fht_beta"
  Sum/1 -> Gain/1
  FHTalpha/1(ualpha) -> Sum/1, Bus Creator/1  "u_fht_alpha"
  abc2alphabeta/2(beta) -> FHTbeta/1(u), Bus Creator1/1  "u_grid_beta"
  abc2alphabeta/1(alpha) -> FHTalpha/1(u), Bus Creator4/1  "u_grid_alpha"
  ug_a/1 -> abc2alphabeta/1(a), grid_voltages/1  "ugd_a"
  ug_c/1 -> abc2alphabeta/3(c), grid_voltages/3  "ugd_c"
  ug_b/1 -> abc2alphabeta/2(b), grid_voltages/2  "ugd_b"

== system afe_dqctrl_inv_psm/afe_dq_mod1/AFE_control/afe_control/grid_voltage_phase_lock_loops/FHT-PLL_simulink/pll_stageA/sequences ==
  u_grid_alpha : Inport
  u_grid_beta : Inport  Port=2
  phase_angle : Inport  Port=3
  alphabeta2xieta : MATLAB Function  TreatAsAtomicUnit=on
  u_grid_xi : Outport
  u_grid_eta : Outport  Port=2
  wires:
  phase_angle/1 -> alphabeta2xieta/3(gamma)  "phase_angle"
  u_grid_beta/1 -> alphabeta2xieta/2(beta)  "u_grid_beta"
  u_grid_alpha/1 -> alphabeta2xieta/1(alpha)  "u_grid_alpha"
  alphabeta2xieta/2(eta) -> u_grid_eta/1  "u_grid_eta"
  alphabeta2xieta/1(xi) -> u_grid_xi/1  "u_grid_xi"
